simulink model "sf_coder_extrinsic_example"  (R2025b)
settings: Solver=VariableStepAuto  StartTime=0.0  StopTime=10.0  RelTol=1e-3
settings Model: Creator=The MathWorks, Inc.  LastModifiedBy=The MathWorks, Inc.
settings SolverCC: AlgebraicLoopSolver=TrustRegion
settings DataIOCC: ReturnWorkspaceOutputs=off
settings OptimizationCC: ReuseModelBlockBuffer=off
settings DebuggingCC: UnconnectedInputMsg=warning  UnconnectedOutputMsg=warning  UnconnectedLineMsg=warning  ArithmeticOperatorsInVariantConditions=warning
settings ModelReferenceCC: EnableRefExpFcnMdlSchedulingChecks=on
settings SFSimCC: SimUseLocalCustomCode=off  CustomCodeUndefinedFunction=UseInterfaceOnly
settings RTWCC: RTWUseLocalCustomCode=off  GPUComputeCapability=3.5
settings CodeAppCC: StateflowObjectComments=on

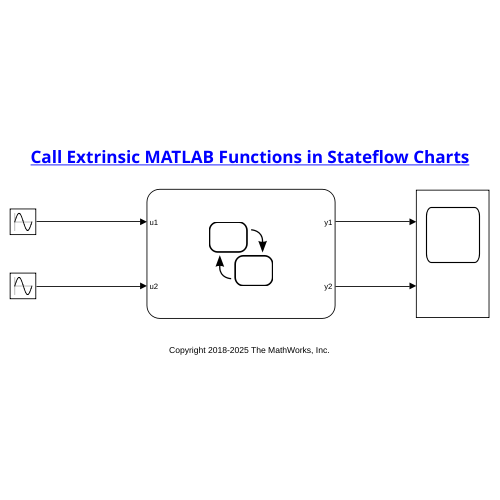
[thumbnail: Simulink's stored preview of the top-level diagram]
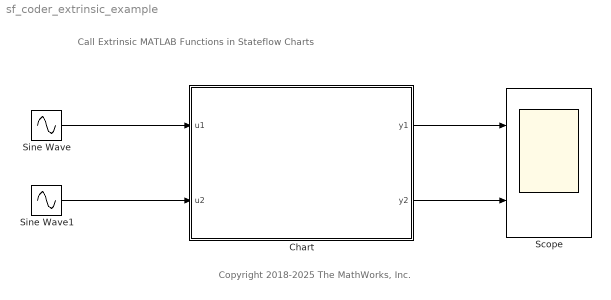
== system sf_coder_extrinsic_example ==
  note: Copyright 2018-2025 The MathWorks, Inc.
  note: Call Extrinsic MATLAB Functions in Stateflow Charts
  Chart : Stateflow chart  TreatAsAtomicUnit=on
  Scope : Scope  NumInputPorts=2
      settings: ActiveDisplayYMinimum=-0.125  ActiveDisplayYMaximum=1.125
  Sine Wave : Sin  SampleTime=0
  Sine Wave1 : Sin  Amplitude=-1  SampleTime=0
  wires:
  Chart/1(y1) -> Scope/1
  Sine Wave/1 -> Chart/1(u1)
  Chart/2(y2) -> Scope/2
  Sine Wave1/1 -> Chart/2(u2)

== stateflow chart sf_coder_extrinsic_example/Chart ==
  state A [parallel]
    en,du:
    coder.extrinsic('heaviside');
    y1 = heaviside(u1);
    settings: executionOrder=1
  state B [parallel]
    settings: executionOrder=2
    state B1
      en,du:
      y2 = heaviside(u2);
    state B2
      en,du:
      y2 = foo(-10);
    (default) -> B1
    B1 -> B2 : [after(5,sec)]{y2 = heaviside(20);}
  state out = foo(in) [function]
    (default) -> (junction 20) : {out = heaviside(in); }
  data: in function_input; out function_output; y1 output =0; u1 input; u2 input; y2 output =0
